simulink model "VCU_Artemiz"  (R2020a)
settings: Solver=FixedStepDiscrete  StartTime=0.0  StopTime=10.0  FixedStep=0.001  RelTol=1e-3  EnableMultiTasking=on
PreLoadFcn:
  | try
  | MDL_setup;
  | catch
  | end
InitFcn:
  | EcoCoder_PreCheckLic();
undefined symbols (not defined in the file): APPS1_max, APPS1_min, APPS2_max, APPS2_min, BRK_TH, DiscIntNeverNeededParam, sigbuilder_block
libraries: CoderSF_BSW_Libs x241, simulink x29
(part 2 of 3)

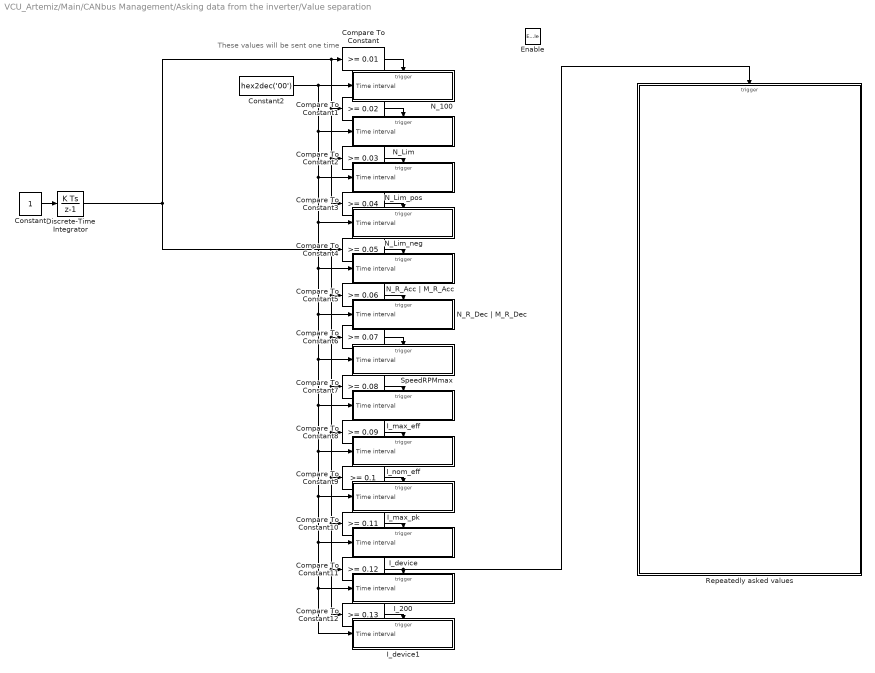
== system VCU_Artemiz/Main/CANbus Management/Asking data from the inverter/Value separation ==
  note: These values will be sent one time
  Enable : EnablePort
  Compare To Constant : simulink/Logic and Bit Operations/Compare To Constant  relop=>=  const=0.01  OutDataTypeStr=boolean
  Compare To Constant1 : simulink/Logic and Bit Operations/Compare To Constant  relop=>=  const=0.02  OutDataTypeStr=boolean
  Compare To Constant10 : simulink/Logic and Bit Operations/Compare To Constant  relop=>=  const=0.11  OutDataTypeStr=boolean
  Compare To Constant11 : simulink/Logic and Bit Operations/Compare To Constant  relop=>=  const=0.12  OutDataTypeStr=boolean
  Compare To Constant12 : simulink/Logic and Bit Operations/Compare To Constant  relop=>=  const=0.13  OutDataTypeStr=boolean
  Compare To Constant2 : simulink/Logic and Bit Operations/Compare To Constant  relop=>=  const=0.03  OutDataTypeStr=boolean
  Compare To Constant3 : simulink/Logic and Bit Operations/Compare To Constant  relop=>=  const=0.04  OutDataTypeStr=boolean
  Compare To Constant4 : simulink/Logic and Bit Operations/Compare To Constant  relop=>=  const=0.05  OutDataTypeStr=boolean
  Compare To Constant5 : simulink/Logic and Bit Operations/Compare To Constant  relop=>=  const=0.06  OutDataTypeStr=boolean
  Compare To Constant6 : simulink/Logic and Bit Operations/Compare To Constant  relop=>=  const=0.07  OutDataTypeStr=boolean
  Compare To Constant7 : simulink/Logic and Bit Operations/Compare To Constant  relop=>=  const=0.08  OutDataTypeStr=boolean
  Compare To Constant8 : simulink/Logic and Bit Operations/Compare To Constant  relop=>=  const=0.09  OutDataTypeStr=boolean
  Compare To Constant9 : simulink/Logic and Bit Operations/Compare To Constant  relop=>=  const=0.1  OutDataTypeStr=boolean
  Constant : Constant  OutDataTypeStr=boolean
  Constant2 : Constant  Value=hex2dec('00')  OutDataTypeStr=uint8
  Discrete-Time Integrator : DiscreteIntegrator  SampleTime=-1  ICPrevOutput=DiscIntNeverNeededParam  ICPrevScaledInput=DiscIntNeverNeededParam
  I_200 : Subsystem
  I_device : Subsystem
  I_device1 : Subsystem
  I_max_eff : Subsystem
  I_max_pk : Subsystem
  I_nom_eff : Subsystem
  N_100 : Subsystem
  N_Lim : Subsystem
  N_Lim_neg : Subsystem
  N_Lim_pos : Subsystem
  N_R_Acc | M_R_Acc : Subsystem
  N_R_Dec | M_R_Dec : Subsystem
  Repeatedly asked values : Subsystem
  SpeedRPMmax : Subsystem
  wires:
  Compare To Constant5/1 -> N_R_Dec | M_R_Dec/Trigger
  Compare To Constant6/1 -> SpeedRPMmax/Trigger
  Compare To Constant4/1 -> N_R_Acc | M_R_Acc/Trigger
  Compare To Constant10/1 -> I_device/Trigger
  Discrete-Time Integrator/1 -> Compare To Constant7/1, Compare To Constant12/1, Compare To Constant11/1, Compare To Constant10/1, Compare To Constant9/1, Compare To Constant8/1, Compare To Constant6/1, Compare To Constant5/1, Compare To Constant4/1, Compare To Constant3/1, Compare To Constant2/1, Compare To Constant1/1, Compare To Constant/1
  Compare To Constant2/1 -> N_Lim_pos/Trigger
  Constant2/1 -> SpeedRPMmax/1(Time interval), I_device1/1(Time interval), I_200/1(Time interval), I_device/1(Time interval), I_max_pk/1(Time interval), I_nom_eff/1(Time interval), I_max_eff/1(Time interval), N_R_Dec | M_R_Dec/1(Time interval), N_R_Acc | M_R_Acc/1(Time interval), N_Lim_neg/1(Time interval), N_Lim_pos/1(Time interval), N_Lim/1(Time interval), N_100/1(Time interval)
  Compare To Constant9/1 -> I_max_pk/Trigger
  Compare To Constant11/1 -> Repeatedly asked values/Trigger, I_200/Trigger
  Compare To Constant/1 -> N_100/Trigger
  Constant/1 -> Discrete-Time Integrator/1
  Compare To Constant7/1 -> I_max_eff/Trigger
  Compare To Constant8/1 -> I_nom_eff/Trigger
  Compare To Constant3/1 -> N_Lim_neg/Trigger
  Compare To Constant1/1 -> N_Lim/Trigger
  Compare To Constant12/1 -> I_device1/Trigger

== system VCU_Artemiz/Main/CANbus Management/Can treatment if len=4 or 5/I_200 ==
  Data : Inport
  Action Port : ActionPort  ActionPortLabel=case [ 217 ]:
  Data Type Conversion : DataTypeConversion
  Write NVM : CoderSF_BSW_Libs/Non-volatile Memory Blocks/Write NVM  variable_name=nvmI_200  flgDef=on  variable_value=0  variable_type=int16  variable_numD=1  unitStr=""  descStr=""  EcoCoderBlockID=N001_NVMVDEF
      settings: AttributesFormatString=value:%<variable_value> type:%<variable_type> D:%<variable_numD>
  Write and Read Measurement : CoderSF_BSW_Libs/Calibration & Measurement/Write and Read Measurement  variable_name=I_200  variable_value=0  variable_type=int16  numD=1  unitStr=""  descStr=""
      settings: AttributesFormatString=type:%<variable_type> Dimensions:%<numD>
  wires:
  Data Type Conversion/1 -> Write and Read Measurement/1
  Write and Read Measurement/1 -> Write NVM/1  "I_200"
  Data/1 -> Data Type Conversion/1

== system VCU_Artemiz/Main/CANbus Management/Can treatment if len=4 or 5/I_act_filt ==
  Data : Inport
  Action Port : ActionPort  ActionPortLabel=case [ 95 ]:
  Data Type Conversion : DataTypeConversion
  Write NVM : CoderSF_BSW_Libs/Non-volatile Memory Blocks/Write NVM  variable_name=nvmI_act_filt  flgDef=on  variable_value=0  variable_type=int16  variable_numD=1  unitStr=""  descStr=""  EcoCoderBlockID=N001_NVMVDEF
      settings: AttributesFormatString=value:%<variable_value> type:%<variable_type> D:%<variable_numD>
  Write and Read Measurement : CoderSF_BSW_Libs/Calibration & Measurement/Write and Read Measurement  variable_name=I_act_filt  variable_value=0  variable_type=int16  numD=1  unitStr=""  descStr=""
      settings: AttributesFormatString=type:%<variable_type> Dimensions:%<numD>
  wires:
  Data Type Conversion/1 -> Write and Read Measurement/1
  Data/1 -> Data Type Conversion/1
  Write and Read Measurement/1 -> Write NVM/1  "I_act_filt"

== system VCU_Artemiz/Main/CANbus Management/Can treatment if len=4 or 5/I_cmd ==
  Data : Inport
  Action Port : ActionPort  ActionPortLabel=case [ 38 ]:
  Data Type Conversion : DataTypeConversion
  Write NVM : CoderSF_BSW_Libs/Non-volatile Memory Blocks/Write NVM  variable_name=nvmI_cmd  flgDef=on  variable_value=0  variable_type=int16  variable_numD=1  unitStr=""  descStr=""  EcoCoderBlockID=N001_NVMVDEF
      settings: AttributesFormatString=value:%<variable_value> type:%<variable_type> D:%<variable_numD>
  Write and Read Measurement : CoderSF_BSW_Libs/Calibration & Measurement/Write and Read Measurement  variable_name=I_cmd  variable_value=0  variable_type=int16  numD=1  unitStr=""  descStr=""
      settings: AttributesFormatString=type:%<variable_type> Dimensions:%<numD>
  wires:
  Data Type Conversion/1 -> Write and Read Measurement/1
  Data/1 -> Data Type Conversion/1
  Write and Read Measurement/1 -> Write NVM/1  "I_cmd"

== system VCU_Artemiz/Main/CANbus Management/Can treatment if len=4 or 5/I_device ==
  Data : Inport
  Action Port : ActionPort  ActionPortLabel=case [ 198 ]:
  Data Type Conversion : DataTypeConversion
  Write NVM : CoderSF_BSW_Libs/Non-volatile Memory Blocks/Write NVM  variable_name=nvmI_device  flgDef=on  variable_value=0  variable_type=int16  variable_numD=1  unitStr=""  descStr=""  EcoCoderBlockID=N001_NVMVDEF
      settings: AttributesFormatString=value:%<variable_value> type:%<variable_type> D:%<variable_numD>
  Write and Read Measurement : CoderSF_BSW_Libs/Calibration & Measurement/Write and Read Measurement  variable_name=I_device  variable_value=0  variable_type=int16  numD=1  unitStr=""  descStr=""
      settings: AttributesFormatString=type:%<variable_type> Dimensions:%<numD>
  wires:
  Data Type Conversion/1 -> Write and Read Measurement/1
  Write and Read Measurement/1 -> Write NVM/1  "I_device"
  Data/1 -> Data Type Conversion/1

== system VCU_Artemiz/Main/CANbus Management/Can treatment if len=4 or 5/I_max_eff ==
  Data : Inport
  Action Port : ActionPort  ActionPortLabel=case [ 77 ]:
  Data Type Conversion : DataTypeConversion
  Write NVM : CoderSF_BSW_Libs/Non-volatile Memory Blocks/Write NVM  variable_name=nvmI_max_eff  flgDef=on  variable_value=0  variable_type=int16  variable_numD=1  unitStr=""  descStr=""  EcoCoderBlockID=N001_NVMVDEF
      settings: AttributesFormatString=value:%<variable_value> type:%<variable_type> D:%<variable_numD>
  Write and Read Measurement : CoderSF_BSW_Libs/Calibration & Measurement/Write and Read Measurement  variable_name=I_max_eff  variable_value=0  variable_type=int16  numD=1  unitStr=""  descStr=""
      settings: AttributesFormatString=type:%<variable_type> Dimensions:%<numD>
  wires:
  Data Type Conversion/1 -> Write and Read Measurement/1
  Data/1 -> Data Type Conversion/1
  Write and Read Measurement/1 -> Write NVM/1  "I_max_eff"

== system VCU_Artemiz/Main/CANbus Management/Can treatment if len=4 or 5/I_max_pk ==
  Data : Inport
  Action Port : ActionPort  ActionPortLabel=case [ 196 ]:
  Data Type Conversion : DataTypeConversion
  Write NVM : CoderSF_BSW_Libs/Non-volatile Memory Blocks/Write NVM  variable_name=nvmI_max_pk  flgDef=on  variable_value=0  variable_type=int16  variable_numD=1  unitStr=""  descStr=""  EcoCoderBlockID=N001_NVMVDEF
      settings: AttributesFormatString=value:%<variable_value> type:%<variable_type> D:%<variable_numD>
  Write and Read Measurement : CoderSF_BSW_Libs/Calibration & Measurement/Write and Read Measurement  variable_name=I_max_pk  variable_value=0  variable_type=int16  numD=1  unitStr=""  descStr=""
      settings: AttributesFormatString=type:%<variable_type> Dimensions:%<numD>
  wires:
  Data Type Conversion/1 -> Write and Read Measurement/1
  Write and Read Measurement/1 -> Write NVM/1  "I_max_pk"
  Data/1 -> Data Type Conversion/1

== system VCU_Artemiz/Main/CANbus Management/Can treatment if len=4 or 5/I_nom_eff ==
  Data : Inport
  Action Port : ActionPort  ActionPortLabel=case [ 78 ]:
  Data Type Conversion : DataTypeConversion
  Write NVM : CoderSF_BSW_Libs/Non-volatile Memory Blocks/Write NVM  variable_name=nvmI_nom_eff  flgDef=on  variable_value=0  variable_type=int16  variable_numD=1  unitStr=""  descStr=""  EcoCoderBlockID=N001_NVMVDEF
      settings: AttributesFormatString=value:%<variable_value> type:%<variable_type> D:%<variable_numD>
  Write and Read Measurement : CoderSF_BSW_Libs/Calibration & Measurement/Write and Read Measurement  variable_name=I_nom_eff  variable_value=0  variable_type=int16  numD=1  unitStr=""  descStr=""
      settings: AttributesFormatString=type:%<variable_type> Dimensions:%<numD>
  wires:
  Data Type Conversion/1 -> Write and Read Measurement/1
  Write and Read Measurement/1 -> Write NVM/1  "I_nom_eff"
  Data/1 -> Data Type Conversion/1

== system VCU_Artemiz/Main/CANbus Management/Can treatment if len=4 or 5/N_100 ==
  Data : Inport
  Action Port : ActionPort  ActionPortLabel=case [ 200 ]:
  Data Type Conversion : DataTypeConversion
  Write NVM : CoderSF_BSW_Libs/Non-volatile Memory Blocks/Write NVM  variable_name=nvmN_100  flgDef=on  variable_value=0  variable_type=uint16  variable_numD=1  unitStr=""  descStr=""  EcoCoderBlockID=N001_NVMVDEF
      settings: AttributesFormatString=value:%<variable_value> type:%<variable_type> D:%<variable_numD>
  Write and Read Measurement : CoderSF_BSW_Libs/Calibration & Measurement/Write and Read Measurement  variable_name=N_100  variable_value=0  variable_type=uint16  numD=1  unitStr=""  descStr=""
      settings: AttributesFormatString=type:%<variable_type> Dimensions:%<numD>
  wires:
  Data Type Conversion/1 -> Write and Read Measurement/1
  Data/1 -> Data Type Conversion/1
  Write and Read Measurement/1 -> Write NVM/1  "N_100"

== system VCU_Artemiz/Main/CANbus Management/Can treatment if len=4 or 5/N_Lim ==
  Data : Inport
  Action Port : ActionPort  ActionPortLabel=case [ 52 ]:
  Data Type Conversion : DataTypeConversion
  Write NVM : CoderSF_BSW_Libs/Non-volatile Memory Blocks/Write NVM  variable_name=nvmN_lim  flgDef=on  variable_value=0  variable_type=uint16  variable_numD=1  unitStr=""  descStr=""  EcoCoderBlockID=N001_NVMVDEF
      settings: AttributesFormatString=value:%<variable_value> type:%<variable_type> D:%<variable_numD>
  Write and Read Measurement : CoderSF_BSW_Libs/Calibration & Measurement/Write and Read Measurement  variable_name=N_lim  variable_value=0  variable_type=uint16  numD=1  unitStr=""  descStr=""
      settings: AttributesFormatString=type:%<variable_type> Dimensions:%<numD>
  wires:
  Data Type Conversion/1 -> Write and Read Measurement/1
  Data/1 -> Data Type Conversion/1
  Write and Read Measurement/1 -> Write NVM/1  "N_lim"

== system VCU_Artemiz/Main/CANbus Management/Can treatment if len=4 or 5/N_Lim_neg ==
  Data : Inport
  Action Port : ActionPort  ActionPortLabel=case [ 62 ]:
  Data Type Conversion : DataTypeConversion
  Write NVM : CoderSF_BSW_Libs/Non-volatile Memory Blocks/Write NVM  variable_name=nvmN_lim_neg  flgDef=on  variable_value=0  variable_type=int16  variable_numD=1  unitStr=""  descStr=""  EcoCoderBlockID=N001_NVMVDEF
      settings: AttributesFormatString=value:%<variable_value> type:%<variable_type> D:%<variable_numD>
  Write and Read Measurement : CoderSF_BSW_Libs/Calibration & Measurement/Write and Read Measurement  variable_name=N_lim_neg  variable_value=0  variable_type=int16  numD=1  unitStr=""  descStr=""
      settings: AttributesFormatString=type:%<variable_type> Dimensions:%<numD>
  wires:
  Data Type Conversion/1 -> Write and Read Measurement/1
  Data/1 -> Data Type Conversion/1
  Write and Read Measurement/1 -> Write NVM/1  "N_lim_neg"

== system VCU_Artemiz/Main/CANbus Management/Can treatment if len=4 or 5/N_Lim_pos ==
  Data : Inport
  Action Port : ActionPort  ActionPortLabel=case [ 63 ]:
  Data Type Conversion : DataTypeConversion
  Write NVM : CoderSF_BSW_Libs/Non-volatile Memory Blocks/Write NVM  variable_name=nvmN_lim_pos  flgDef=on  variable_value=0  variable_type=int16  variable_numD=1  unitStr=""  descStr=""  EcoCoderBlockID=N001_NVMVDEF
      settings: AttributesFormatString=value:%<variable_value> type:%<variable_type> D:%<variable_numD>
  Write and Read Measurement : CoderSF_BSW_Libs/Calibration & Measurement/Write and Read Measurement  variable_name=N_lim_pos  variable_value=0  variable_type=int16  numD=1  unitStr=""  descStr=""
      settings: AttributesFormatString=type:%<variable_type> Dimensions:%<numD>
  wires:
  Data Type Conversion/1 -> Write and Read Measurement/1
  Data/1 -> Data Type Conversion/1
  Write and Read Measurement/1 -> Write NVM/1  "N_lim_pos"

== system VCU_Artemiz/Main/CANbus Management/Can treatment if len=4 or 5/N_act_filt ==
  Data : Inport
  Action Port : ActionPort  ActionPortLabel=case [ 168 ]:
  Data Type Conversion : DataTypeConversion
  Write NVM : CoderSF_BSW_Libs/Non-volatile Memory Blocks/Write NVM  variable_name=nvmN_act_filt  flgDef=on  variable_value=0  variable_type=int16  variable_numD=1  unitStr=""  descStr=""  EcoCoderBlockID=N001_NVMVDEF
      settings: AttributesFormatString=value:%<variable_value> type:%<variable_type> D:%<variable_numD>
  Write and Read Measurement : CoderSF_BSW_Libs/Calibration & Measurement/Write and Read Measurement  variable_name=N_act_filt  variable_value=0  variable_type=int16  numD=1  unitStr=""  descStr=""
      settings: AttributesFormatString=type:%<variable_type> Dimensions:%<numD>
  wires:
  Data Type Conversion/1 -> Write and Read Measurement/1
  Write and Read Measurement/1 -> Write NVM/1  "N_act_filt"
  Data/1 -> Data Type Conversion/1

== system VCU_Artemiz/Main/CANbus Management/Can treatment if len=4 or 5/SpeedRPMmax ==
  Data : Inport
  Action Port : ActionPort  ActionPortLabel=case [ 206 ]:
  Data Type Conversion : DataTypeConversion
  Write NVM : CoderSF_BSW_Libs/Non-volatile Memory Blocks/Write NVM  variable_name=nvmSpeedRPMmax  flgDef=on  variable_value=0  variable_type=int16  variable_numD=1  unitStr=""  descStr=""  EcoCoderBlockID=N001_NVMVDEF
      settings: AttributesFormatString=value:%<variable_value> type:%<variable_type> D:%<variable_numD>
  Write and Read Measurement : CoderSF_BSW_Libs/Calibration & Measurement/Write and Read Measurement  variable_name=SpeedRPMmax  variable_value=0  variable_type=int16  numD=1  unitStr=""  descStr=""
      settings: AttributesFormatString=type:%<variable_type> Dimensions:%<numD>
  wires:
  Data Type Conversion/1 -> Write and Read Measurement/1
  Write and Read Measurement/1 -> Write NVM/1  "SpeedRPMmax"
  Data/1 -> Data Type Conversion/1

== system VCU_Artemiz/Main/CANbus Management/Can treatment if len=4 or 5/T_IGBT ==
  Data : Inport
  Action Port : ActionPort  ActionPortLabel=case [ 74 ]:
  Data Type Conversion : DataTypeConversion
  Write NVM : CoderSF_BSW_Libs/Non-volatile Memory Blocks/Write NVM  variable_name=nvmT_IGBT  flgDef=on  variable_value=0  variable_type=int16  variable_numD=1  unitStr=""  descStr=""  EcoCoderBlockID=N001_NVMVDEF
      settings: AttributesFormatString=value:%<variable_value> type:%<variable_type> D:%<variable_numD>
  Write and Read Measurement : CoderSF_BSW_Libs/Calibration & Measurement/Write and Read Measurement  variable_name=T_IGBT  variable_value=0  variable_type=int16  numD=1  unitStr=""  descStr=""
      settings: AttributesFormatString=type:%<variable_type> Dimensions:%<numD>
  wires:
  Data Type Conversion/1 -> Write and Read Measurement/1
  Data/1 -> Data Type Conversion/1
  Write and Read Measurement/1 -> Write NVM/1  "T_IGBT"

== system VCU_Artemiz/Main/CANbus Management/Can treatment if len=4 or 5/T_air ==
  Data : Inport
  Action Port : ActionPort  ActionPortLabel=case [ 75 ]:
  Data Type Conversion : DataTypeConversion
  Write NVM : CoderSF_BSW_Libs/Non-volatile Memory Blocks/Write NVM  variable_name=nvmT_air  flgDef=on  variable_value=0  variable_type=int16  variable_numD=1  unitStr=""  descStr=""  EcoCoderBlockID=N001_NVMVDEF
      settings: AttributesFormatString=value:%<variable_value> type:%<variable_type> D:%<variable_numD>
  Write and Read Measurement : CoderSF_BSW_Libs/Calibration & Measurement/Write and Read Measurement  variable_name=T_air  variable_value=0  variable_type=int16  numD=1  unitStr=""  descStr=""
      settings: AttributesFormatString=type:%<variable_type> Dimensions:%<numD>
  wires:
  Data Type Conversion/1 -> Write and Read Measurement/1
  Data/1 -> Data Type Conversion/1
  Write and Read Measurement/1 -> Write NVM/1  "T_air"

== system VCU_Artemiz/Main/CANbus Management/Can treatment if len=4 or 5/T_motor ==
  Data : Inport
  Action Port : ActionPort  ActionPortLabel=case [ 73 ]:
  Data Type Conversion : DataTypeConversion
  Write NVM : CoderSF_BSW_Libs/Non-volatile Memory Blocks/Write NVM  variable_name=nvmT_motor  flgDef=on  variable_value=0  variable_type=int16  variable_numD=1  unitStr=""  descStr=""  EcoCoderBlockID=N001_NVMVDEF
      settings: AttributesFormatString=value:%<variable_value> type:%<variable_type> D:%<variable_numD>
  Write and Read Measurement : CoderSF_BSW_Libs/Calibration & Measurement/Write and Read Measurement  variable_name=T_motor  variable_value=0  variable_type=int16  numD=1  unitStr=""  descStr=""
      settings: AttributesFormatString=type:%<variable_type> Dimensions:%<numD>
  wires:
  Data Type Conversion/1 -> Write and Read Measurement/1
  Data/1 -> Data Type Conversion/1
  Write and Read Measurement/1 -> Write NVM/1  "T_motor"

== system VCU_Artemiz/Main/CANbus Management/Can treatment if len=4 or 5/Vdc_bus ==
  Data : Inport
  Action Port : ActionPort  ActionPortLabel=case [ 235 ]:
  Data Type Conversion : DataTypeConversion
  Write NVM : CoderSF_BSW_Libs/Non-volatile Memory Blocks/Write NVM  variable_name=nvmVdc_bus  flgDef=on  variable_value=0  variable_type=int16  variable_numD=1  unitStr=""  descStr=""  EcoCoderBlockID=N001_NVMVDEF
      settings: AttributesFormatString=value:%<variable_value> type:%<variable_type> D:%<variable_numD>
  Write and Read Measurement : CoderSF_BSW_Libs/Calibration & Measurement/Write and Read Measurement  variable_name=Vdc_bus  variable_value=0  variable_type=int16  numD=1  unitStr=""  descStr=""
      settings: AttributesFormatString=type:%<variable_type> Dimensions:%<numD>
  wires:
  Data Type Conversion/1 -> Write and Read Measurement/1
  Data/1 -> Data Type Conversion/1
  Write and Read Measurement/1 -> Write NVM/1  "Vdc_bus"

== system VCU_Artemiz/Main/CANbus Management/Can treatment if len=6/N_R_Acc | M R_Acc ==
  Data : Inport
  Action Port : ActionPort  ActionPortLabel=case [ 53 ]:
  Data Type Conversion1 : DataTypeConversion  OutDataTypeStr=int16
  Data Type Conversion2 : DataTypeConversion  OutDataTypeStr=int16
  Extract Bits : simulink/Logic and Bit Operations/Extract Bits  bitsToExtract=Lower half  numBits=8  bitIdxRange=[0 7]  outScalingMode=Treat bit field as an integer
  Extract Bits1 : simulink/Logic and Bit Operations/Extract Bits  bitsToExtract=Upper half  numBits=8  bitIdxRange=[0 7]  outScalingMode=Treat bit field as an integer
  Write NVM : CoderSF_BSW_Libs/Non-volatile Memory Blocks/Write NVM  variable_name=nvmN_R_Acc  flgDef=on  variable_value=0  variable_type=int16  variable_numD=1  unitStr=""  descStr=""  EcoCoderBlockID=N001_NVMVDEF
      settings: AttributesFormatString=value:%<variable_value> type:%<variable_type> D:%<variable_numD>
  Write NVM1 : CoderSF_BSW_Libs/Non-volatile Memory Blocks/Write NVM  variable_name=nvmM_R_Acc  flgDef=on  variable_value=0  variable_type=int16  variable_numD=1  unitStr=""  descStr=""  EcoCoderBlockID=N001_NVMVDEF
      settings: AttributesFormatString=value:%<variable_value> type:%<variable_type> D:%<variable_numD>
  Write and Read Measurement : CoderSF_BSW_Libs/Calibration & Measurement/Write and Read Measurement  variable_name=N_R_Acc  variable_value=0  variable_type=int16  numD=1  unitStr=""  descStr=""
      settings: AttributesFormatString=type:%<variable_type> Dimensions:%<numD>
  Write and Read Measurement1 : CoderSF_BSW_Libs/Calibration & Measurement/Write and Read Measurement  variable_name=M_R_Acc  variable_value=0  variable_type=int16  numD=1  unitStr=""  descStr=""
      settings: AttributesFormatString=type:%<variable_type> Dimensions:%<numD>
  wires:
  Data/1 -> Extract Bits1/1, Extract Bits/1
  Extract Bits/1 -> Data Type Conversion2/1
  Data Type Conversion2/1 -> Write and Read Measurement/1
  Extract Bits1/1 -> Data Type Conversion1/1
  Data Type Conversion1/1 -> Write and Read Measurement1/1
  Write and Read Measurement/1 -> Write NVM/1  "N_R_Acc"
  Write and Read Measurement1/1 -> Write NVM1/1  "M_R_Acc"

== system VCU_Artemiz/Main/CANbus Management/Can treatment if len=6/N_R_Dec | M_R_Dec ==
  Data : Inport
  Action Port : ActionPort  ActionPortLabel=case [ 237 ]:
  Data Type Conversion1 : DataTypeConversion  OutDataTypeStr=int16
  Data Type Conversion2 : DataTypeConversion  OutDataTypeStr=int16
  Extract Bits : simulink/Logic and Bit Operations/Extract Bits  bitsToExtract=Lower half  numBits=8  bitIdxRange=[0 7]  outScalingMode=Treat bit field as an integer
  Extract Bits1 : simulink/Logic and Bit Operations/Extract Bits  bitsToExtract=Upper half  numBits=8  bitIdxRange=[0 7]  outScalingMode=Treat bit field as an integer
  Write NVM : CoderSF_BSW_Libs/Non-volatile Memory Blocks/Write NVM  variable_name=nvmN_R_Dec  flgDef=on  variable_value=0  variable_type=int16  variable_numD=1  unitStr=""  descStr=""  EcoCoderBlockID=N001_NVMVDEF
      settings: AttributesFormatString=value:%<variable_value> type:%<variable_type> D:%<variable_numD>
  Write NVM1 : CoderSF_BSW_Libs/Non-volatile Memory Blocks/Write NVM  variable_name=nvmM_R_Dec  flgDef=on  variable_value=0  variable_type=int16  variable_numD=1  unitStr=""  descStr=""  EcoCoderBlockID=N001_NVMVDEF
      settings: AttributesFormatString=value:%<variable_value> type:%<variable_type> D:%<variable_numD>
  Write and Read Measurement : CoderSF_BSW_Libs/Calibration & Measurement/Write and Read Measurement  variable_name=N_R_Dec  variable_value=0  variable_type=int16  numD=1  unitStr=""  descStr=""
      settings: AttributesFormatString=type:%<variable_type> Dimensions:%<numD>
  Write and Read Measurement1 : CoderSF_BSW_Libs/Calibration & Measurement/Write and Read Measurement  variable_name=M_R_Dec  variable_value=0  variable_type=int16  numD=1  unitStr=""  descStr=""
      settings: AttributesFormatString=type:%<variable_type> Dimensions:%<numD>
  wires:
  Data Type Conversion2/1 -> Write and Read Measurement/1
  Data Type Conversion1/1 -> Write and Read Measurement1/1
  Data/1 -> Extract Bits1/1, Extract Bits/1
  Extract Bits1/1 -> Data Type Conversion1/1
  Extract Bits/1 -> Data Type Conversion2/1
  Write and Read Measurement/1 -> Write NVM/1  "N_R_Dec"
  Write and Read Measurement1/1 -> Write NVM1/1  "M_R_Dec"

== system VCU_Artemiz/Main/CANbus Management/Initialization/Disabling the inverter ==
  Constant : Constant  Value=hex2dec('51')  OutDataTypeStr=uint8
  Constant1 : Constant  Value=hex2dec('0004')  OutDataTypeStr=uint16
  Pack Signals To CAN Data : CoderSF_BSW_Libs/CAN/Pack Signals To CAN Data  Signal="{{'REG_ID'  'Data1'},[0 8],[8 16],{'uint8'  'uint16'},{'Intel' 'Intel'}}"
  Send CAN Data : CoderSF_BSW_Libs/CAN/Send CAN Data  channel=CAN_A  txlen=3  txid=hex2dec('201')  frametype=Standard(11-bit ID)  showerror=off
  wires:
  Constant/1 -> Pack Signals To CAN Data/1
  Pack Signals To CAN Data/1 -> Send CAN Data/1
  Constant1/1 -> Pack Signals To CAN Data/2

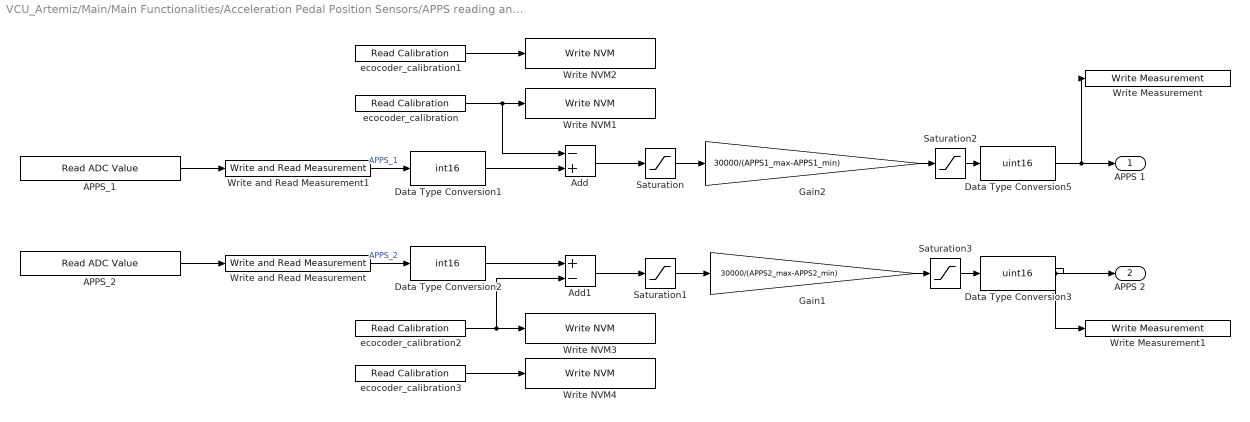
== system VCU_Artemiz/Main/Main Functionalities/Acceleration Pedal Position Sensors/APPS reading and calibration ==
  APPS_1 : CoderSF_BSW_Libs/ADC/Read ADC Value  channel=3
  APPS_2 : CoderSF_BSW_Libs/ADC/Read ADC Value  channel=4
  Add : Sum  Inputs=-+
  Add1 : Sum  Inputs=+-
  Data Type Conversion1 : DataTypeConversion  OutDataTypeStr=int16
  Data Type Conversion2 : DataTypeConversion  OutDataTypeStr=int16
  Data Type Conversion3 : DataTypeConversion  OutDataTypeStr=uint16
  Data Type Conversion5 : DataTypeConversion  OutDataTypeStr=uint16
  Gain1 : Gain  Gain=30000/(APPS2_max-APPS2_min)  OutDataTypeStr=int32
  Gain2 : Gain  Gain=30000/(APPS1_max-APPS1_min)  OutDataTypeStr=int32
  Saturation : Saturate  UpperLimit=4095  LowerLimit=0  OutDataTypeStr=int16
  Saturation1 : Saturate  UpperLimit=4095  LowerLimit=0  OutDataTypeStr=int16
  Saturation2 : Saturate  UpperLimit=30000  LowerLimit=0  OutDataTypeStr=int32
  Saturation3 : Saturate  UpperLimit=30000  LowerLimit=0  OutDataTypeStr=int32
  Write Measurement : CoderSF_BSW_Libs/Calibration & Measurement/Write Measurement  variable_name=APPS1_calib  variable_value=0  variable_type=uint16  numD=1  unitStr=""  descStr=""
      settings: AttributesFormatString=type:%<variable_type> Dimensions:%<numD>
  Write Measurement1 : CoderSF_BSW_Libs/Calibration & Measurement/Write Measurement  variable_name=APPS2_calib  variable_value=0  variable_type=uint16  numD=1  unitStr=""  descStr=""
      settings: AttributesFormatString=type:%<variable_type> Dimensions:%<numD>
  Write NVM1 : CoderSF_BSW_Libs/Non-volatile Memory Blocks/Write NVM  variable_name=nvmAPPS1_min  flgDef=on  variable_value=0  variable_type=int16  variable_numD=1  unitStr=""  descStr=""  EcoCoderBlockID=N001_NVMVDEF
      settings: AttributesFormatString=value:%<variable_value> type:%<variable_type> D:%<variable_numD>
  Write NVM2 : CoderSF_BSW_Libs/Non-volatile Memory Blocks/Write NVM  variable_name=nvmAPPS1_max  flgDef=on  variable_value=0  variable_type=int16  variable_numD=1  unitStr=""  descStr=""  EcoCoderBlockID=N001_NVMVDEF
      settings: AttributesFormatString=value:%<variable_value> type:%<variable_type> D:%<variable_numD>
  Write NVM3 : CoderSF_BSW_Libs/Non-volatile Memory Blocks/Write NVM  variable_name=nvmAPPS2_min  flgDef=on  variable_value=0  variable_type=int16  variable_numD=1  unitStr=""  descStr=""  EcoCoderBlockID=N001_NVMVDEF
      settings: AttributesFormatString=value:%<variable_value> type:%<variable_type> D:%<variable_numD>
  Write NVM4 : CoderSF_BSW_Libs/Non-volatile Memory Blocks/Write NVM  variable_name=nvmAPPS2_max  flgDef=on  variable_value=0  variable_type=int16  variable_numD=1  unitStr=""  descStr=""  EcoCoderBlockID=N001_NVMVDEF
      settings: AttributesFormatString=value:%<variable_value> type:%<variable_type> D:%<variable_numD>
  Write and Read Measurement : CoderSF_BSW_Libs/Calibration & Measurement/Write and Read Measurement  variable_name=APPS_2  variable_value=0  variable_type=uint16  numD=1  unitStr=""  descStr=""
      settings: AttributesFormatString=type:%<variable_type> Dimensions:%<numD>
  Write and Read Measurement1 : CoderSF_BSW_Libs/Calibration & Measurement/Write and Read Measurement  variable_name=APPS_1  variable_value=0  variable_type=uint16  numD=1  unitStr=""  descStr=""
      settings: AttributesFormatString=type:%<variable_type> Dimensions:%<numD>
  ecocoder_calibration : CoderSF_BSW_Libs/Calibration & Measurement/Read Calibration  variable_name=APPS1_min  variable_value=750  variable_type=int16  variable_min=[]  variable_max=[]  unitStr=""  descStr=""
      settings: AttributesFormatString=value:%<variable_value> type:%<variable_type> max:%<variable_max> Min:%<variable_min>
  ecocoder_calibration1 : CoderSF_BSW_Libs/Calibration & Measurement/Read Calibration  variable_name=APPS1_max  variable_value=1293  variable_type=int16  variable_min=[]  variable_max=[]  unitStr=""  descStr=""
      settings: AttributesFormatString=value:%<variable_value> type:%<variable_type> max:%<variable_max> Min:%<variable_min>
  ecocoder_calibration2 : CoderSF_BSW_Libs/Calibration & Measurement/Read Calibration  variable_name=APPS2_min  variable_value=366  variable_type=int16  variable_min=[]  variable_max=[]  unitStr=""  descStr=""
      settings: AttributesFormatString=value:%<variable_value> type:%<variable_type> max:%<variable_max> Min:%<variable_min>
  ecocoder_calibration3 : CoderSF_BSW_Libs/Calibration & Measurement/Read Calibration  variable_name=APPS2_max  variable_value=912  variable_type=int16  variable_min=[]  variable_max=[]  unitStr=""  descStr=""
      settings: AttributesFormatString=value:%<variable_value> type:%<variable_type> max:%<variable_max> Min:%<variable_min>
  APPS 1 : Outport
  APPS 2 : Outport  Port=2
  wires:
  APPS_2/1 -> Write and Read Measurement/1
  Write and Read Measurement1/1 -> Data Type Conversion1/1  "APPS_1"
  Write and Read Measurement/1 -> Data Type Conversion2/1  "APPS_2"
  APPS_1/1 -> Write and Read Measurement1/1
  Saturation/1 -> Gain2/1
  Data Type Conversion5/1 -> Write Measurement/1, APPS 1/1
  ecocoder_calibration/1 -> Add/1, Write NVM1/1
  ecocoder_calibration1/1 -> Write NVM2/1
  ecocoder_calibration2/1 -> Add1/2, Write NVM3/1
  ecocoder_calibration3/1 -> Write NVM4/1
  Data Type Conversion1/1 -> Add/2
  Add/1 -> Saturation/1
  Add1/1 -> Saturation1/1
  Saturation1/1 -> Gain1/1
  Data Type Conversion3/1 -> Write Measurement1/1, APPS 2/1
  Data Type Conversion2/1 -> Add1/1
  Gain2/1 -> Saturation2/1
  Saturation2/1 -> Data Type Conversion5/1
  Gain1/1 -> Saturation3/1
  Saturation3/1 -> Data Type Conversion3/1

== system VCU_Artemiz/Main/Main Functionalities/Acceleration Pedal Position Sensors/Check APPS Implausibility ==
  note: Check if the implausibility persists for more than 100ms
  note: Check if there is an APPS implausibility (T 11.8.9)
  APPS 1 : Inport
  APPS 2 : Inport  Port=2
  Abs : Abs  OutDataTypeStr=uint16
  Compare To Constant : simulink/Logic and Bit Operations/Compare To Constant  relop=>=  const=30000  OutDataTypeStr=boolean
  Compare To Constant1 : simulink/Logic and Bit Operations/Compare To Constant  relop=>=  const=0.1  OutDataTypeStr=boolean
  Discrete-Time Integrator : DiscreteIntegrator  ExternalReset=falling  SampleTime=-1  OutDataTypeStr=Inherit: Inherit via back propagation  UpperSaturationLimit=12  ICPrevOutput=DiscIntNeverNeededParam  ICPrevScaledInput=DiscIntNeverNeededParam
  Gain1 : Gain  Gain=10  OutDataTypeStr=uint32
  Subtract : Sum  Inputs=+-  OutDataTypeStr=int16
  Write Measurement : CoderSF_BSW_Libs/Calibration & Measurement/Write Measurement  variable_name=APPS_PBM  variable_value=0  variable_type=boolean  numD=1  unitStr=""  descStr=""
      settings: AttributesFormatString=type:%<variable_type> Dimensions:%<numD>
  Write Measurement2 : CoderSF_BSW_Libs/Calibration & Measurement/Write Measurement  variable_name=APPS_implausibility  variable_value=0  variable_type=boolean  numD=1  unitStr=""  descStr=""
      settings: AttributesFormatString=type:%<variable_type> Dimensions:%<numD>
  Write NVM4 : CoderSF_BSW_Libs/Non-volatile Memory Blocks/Write NVM  variable_name=nvmAPPS_PBM  flgDef=on  variable_value=0  variable_type=boolean  variable_numD=1  unitStr=""  descStr=""  EcoCoderBlockID=N001_NVMVDEF
      settings: AttributesFormatString=value:%<variable_value> type:%<variable_type> D:%<variable_numD>
  tag scope: APPS_PBM=global
  wires:
  Discrete-Time Integrator/1 -> Compare To Constant1/1
  Subtract/1 -> Abs/1
  Compare To Constant/1 -> Write Measurement2/1, Discrete-Time Integrator/2, Discrete-Time Integrator/1
  APPS 2/1 -> Subtract/2
  Abs/1 -> Gain1/1
  Compare To Constant1/1 -> [APPS_PBM], Write Measurement/1, Write NVM4/1  "APPS_PBM"
  Gain1/1 -> Compare To Constant/1
  APPS 1/1 -> Subtract/1

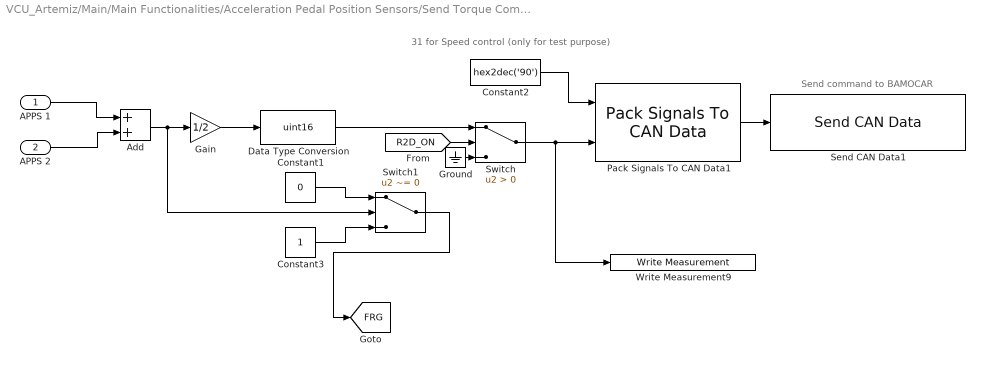
== system VCU_Artemiz/Main/Main Functionalities/Acceleration Pedal Position Sensors/Send Torque Command ==
  note: 31 for Speed control (only for test purpose)
  note: Send command to BAMOCAR
  APPS 1 : Inport
  APPS 2 : Inport  Port=2
  Add : Sum  OutDataTypeStr=uint32
  Constant1 : Constant  Value=0  OutDataTypeStr=boolean
  Constant2 : Constant  Value=hex2dec('90')  OutDataTypeStr=uint8
  Constant3 : Constant  OutDataTypeStr=boolean
  Data Type Conversion : DataTypeConversion  OutDataTypeStr=uint16
  Gain : Gain  Gain=1/2
  Ground : Ground
  Pack Signals To CAN Data1 : CoderSF_BSW_Libs/CAN/Pack Signals To CAN Data  Signal="{{'REG_90'  'Data1'},[0 8],[8 24],{'uint8'  'uint16'},{'Intel' 'Intel'}}"
  Send CAN Data1 : CoderSF_BSW_Libs/CAN/Send CAN Data  channel=CAN_A  txlen=3  txid="hex2dec(\"201\")"  frametype=Standard(11-bit ID)  showerror=off
  Switch : Switch  Criteria=u2 > Threshold
  Switch1 : Switch  Criteria=u2 ~= 0  Threshold=1
  Write Measurement9 : CoderSF_BSW_Libs/Calibration & Measurement/Write Measurement  variable_name=TRQ_CMD_BAMOCAR  variable_value=0  variable_type=uint16  numD=1  unitStr=""  descStr=""
      settings: AttributesFormatString=type:%<variable_type> Dimensions:%<numD>
  tag scope: FRG=global
  wires:
  Pack Signals To CAN Data1/1 -> Send CAN Data1/1
  Gain/1 -> Data Type Conversion/1
  APPS 2/1 -> Add/2
  APPS 1/1 -> Add/1
  Constant2/1 -> Pack Signals To CAN Data1/1
  [R2D_ON] -> Switch/2
  Switch/1 -> Write Measurement9/1, Pack Signals To CAN Data1/2
  Ground/1 -> Switch/3
  Data Type Conversion/1 -> Switch/1
  Add/1 -> Switch1/2, Gain/1
  Constant1/1 -> Switch1/1
  Constant3/1 -> Switch1/3
  Switch1/1 -> [FRG]

== system VCU_Artemiz/Main/Main Functionalities/Ready to drive/Enable Inverter ==
  Trigger : TriggerPort  TriggerType=either  VariantControl=Variant  PortDimensions=1
  Constant : Constant  Value=hex2dec('51')  OutDataTypeStr=uint8
  Constant1 : Constant  Value=hex2dec('0000')  OutDataTypeStr=uint16
  Pack Signals To CAN Data : CoderSF_BSW_Libs/CAN/Pack Signals To CAN Data  Signal="{{'REG_ID'  'Data1'},[0 8],[8 16],{'uint8'  'uint16'},{'Intel' 'Intel'}}"
  Send CAN Data : CoderSF_BSW_Libs/CAN/Send CAN Data  channel=CAN_A  txlen=3  txid=hex2dec('201')  frametype=Standard(11-bit ID)  showerror=off
  wires:
  Constant/1 -> Pack Signals To CAN Data/1
  Pack Signals To CAN Data/1 -> Send CAN Data/1
  Constant1/1 -> Pack Signals To CAN Data/2

== system VCU_Artemiz/Main/Main Functionalities/Ready to drive/Subsystem ==
  note: Must press during 1s
  Compare To Constant3 : simulink/Logic and Bit Operations/Compare To Constant  relop=>=  const=1  OutDataTypeStr=boolean
  Discrete-Time Integrator1 : DiscreteIntegrator  ExternalReset=falling  SampleTime=-1  OutDataTypeStr=Inherit: Inherit via back propagation  UpperSaturationLimit=12  ICPrevOutput=DiscIntNeverNeededParam  ICPrevScaledInput=DiscIntNeverNeededParam
  FLWS : CoderSF_BSW_Libs/Digital I//O/Switch Input  portNum=DI32
  Logical Operator : Logic  AllPortsSameDT=off  OutDataTypeStr=boolean
  R2D Button : CoderSF_BSW_Libs/Digital I//O/Switch Input  portNum=DI13
  Write Measurement1 : CoderSF_BSW_Libs/Calibration & Measurement/Write Measurement  variable_name=FLWS  variable_value=0  variable_type=boolean  numD=1  unitStr=""  descStr=""
      settings: AttributesFormatString=type:%<variable_type> Dimensions:%<numD>
  Write Measurement6 : CoderSF_BSW_Libs/Calibration & Measurement/Write Measurement  variable_name=R2D_btn  variable_value=0  variable_type=boolean  numD=1  unitStr=""  descStr=""
      settings: AttributesFormatString=type:%<variable_type> Dimensions:%<numD>
  R2D_ASKED : Outport
  wires:
  Logical Operator/1 -> Discrete-Time Integrator1/1, Discrete-Time Integrator1/2
  Discrete-Time Integrator1/1 -> Compare To Constant3/1
  [BRAKE_ON] -> Logical Operator/1
  Compare To Constant3/1 -> R2D_ASKED/1
  R2D Button/1 -> Logical Operator/2, Write Measurement6/1
  FLWS/1 -> Write Measurement1/1

== system VCU_Artemiz/Main/Main Functionalities/Ready to drive/Subsystem1 ==
  Trigger : Inport
  Exit : Inport  Port=2
  Compare To Constant5 : simulink/Logic and Bit Operations/Compare To Constant  relop=<=  const=2  OutDataTypeStr=boolean
  Compare To Constant7 : simulink/Logic and Bit Operations/Compare To Constant  relop=>  const=0.1  OutDataTypeStr=boolean
  Discrete-Time Integrator2 : DiscreteIntegrator  ExternalReset=falling  SampleTime=-1  OutDataTypeStr=Inherit: Inherit via back propagation  UpperSaturationLimit=12  ICPrevOutput=DiscIntNeverNeededParam  ICPrevScaledInput=DiscIntNeverNeededParam
  Enter R2D Mode : Subsystem  TreatAsAtomicUnit=on
  Logical Operator5 : Logic  IconShape=distinctive  AllPortsSameDT=off  OutDataTypeStr=boolean
  R2D LED : CoderSF_BSW_Libs/Digital I//O/Switch Output  channel=LSO03
  R2D Sound : CoderSF_BSW_Libs/Digital I//O/Switch Output  channel=LSO01
  Write Measurement : CoderSF_BSW_Libs/Calibration & Measurement/Write Measurement  variable_name=R2D  variable_value=0  variable_type=boolean  numD=1  unitStr=""  descStr=""
      settings: AttributesFormatString=type:%<variable_type> Dimensions:%<numD>
  Write Measurement3 : CoderSF_BSW_Libs/Calibration & Measurement/Write Measurement  variable_name=BUZZ  variable_value=0  variable_type=boolean  numD=1  unitStr=""  descStr=""
      settings: AttributesFormatString=type:%<variable_type> Dimensions:%<numD>
  Write NVM : CoderSF_BSW_Libs/Non-volatile Memory Blocks/Write NVM  variable_name=nvm_R2D  flgDef=on  variable_value=0  variable_type=boolean  variable_numD=1  unitStr=""  descStr=""  EcoCoderBlockID=N001_NVMVDEF
      settings: AttributesFormatString=value:%<variable_value> type:%<variable_type> D:%<variable_numD>
  tag scope: R2D_ON=global
  wires:
  Trigger/1 -> Enter R2D Mode/Trigger
  Exit/1 -> Enter R2D Mode/1(Exit)
  Compare To Constant5/1 -> Logical Operator5/2
  Compare To Constant7/1 -> Logical Operator5/1
  Enter R2D Mode/1(R2D Sound) -> Discrete-Time Integrator2/1, Discrete-Time Integrator2/2
  Discrete-Time Integrator2/1 -> Compare To Constant7/1, Compare To Constant5/1
  Logical Operator5/1 -> R2D Sound/1, Write Measurement3/1
  Enter R2D Mode/2(R2D Led) -> R2D LED/1, Write NVM/1, Write Measurement/1, [R2D_ON]

== system VCU_Artemiz/Main/Main Functionalities/Tractive System/Subsystem ==
  note: Must press during 1s
  Compare To Constant3 : simulink/Logic and Bit Operations/Compare To Constant  relop=>=  const=1  OutDataTypeStr=boolean
  Discrete-Time Integrator1 : DiscreteIntegrator  ExternalReset=falling  SampleTime=-1  OutDataTypeStr=Inherit: Inherit via back propagation  UpperSaturationLimit=12  ICPrevOutput=DiscIntNeverNeededParam  ICPrevScaledInput=DiscIntNeverNeededParam
  Pump2 : CoderSF_BSW_Libs/Digital I//O/Switch Output  channel=LSO06
  Subsystem : Subsystem
  TS Button : CoderSF_BSW_Libs/Digital I//O/Switch Input  portNum=DI09
  Write Measurement : CoderSF_BSW_Libs/Calibration & Measurement/Write Measurement  variable_name=TS  variable_value=0  variable_type=boolean  numD=1  unitStr=""  descStr=""
      settings: AttributesFormatString=type:%<variable_type> Dimensions:%<numD>
  Write Measurement1 : CoderSF_BSW_Libs/Calibration & Measurement/Write Measurement  variable_name=TSBTN  variable_value=0  variable_type=boolean  numD=1  unitStr=""  descStr=""
      settings: AttributesFormatString=type:%<variable_type> Dimensions:%<numD>
  Write NVM : CoderSF_BSW_Libs/Non-volatile Memory Blocks/Write NVM  variable_name=nvm_TS_ON  flgDef=on  variable_value=false  variable_type=boolean  variable_numD=1  unitStr=""  descStr=""  EcoCoderBlockID=N001_NVMVDEF
      settings: AttributesFormatString=value:%<variable_value> type:%<variable_type> D:%<variable_numD>
  TS ON : Outport
  tag scope: TS_ON=global
  wires:
  Discrete-Time Integrator1/1 -> Compare To Constant3/1
  Compare To Constant3/1 -> Subsystem/Trigger, Subsystem/1(In1)
  Subsystem/1(TS ON) -> Write Measurement/1, Write NVM/1, Pump2/1, TS ON/1, [TS_ON]
  TS Button/1 -> Discrete-Time Integrator1/1, Discrete-Time Integrator1/2, Write Measurement1/1

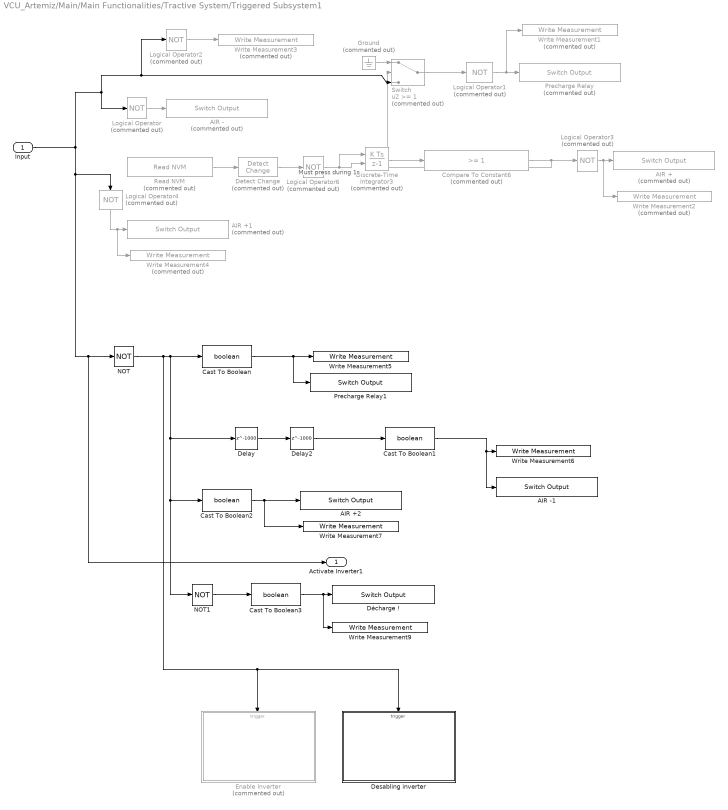
== system VCU_Artemiz/Main/Main Functionalities/Tractive System/Triggered Subsystem1 ==
  note: Must press during 1s
  Input : Inport
  AIR + : CoderSF_BSW_Libs/Digital I//O/Switch Output  Commented=on  channel=HSO03
  AIR +1 : CoderSF_BSW_Libs/Digital I//O/Switch Output  Commented=on  channel=HSO03
  AIR +2 : CoderSF_BSW_Libs/Digital I//O/Switch Output  channel=HSO04
  AIR - : CoderSF_BSW_Libs/Digital I//O/Switch Output  Commented=on  channel=HSO04
  AIR -1 : CoderSF_BSW_Libs/Digital I//O/Switch Output  channel=HSO03
  Cast To Boolean{,1..3} (4 alike) : DataTypeConversion  OutDataTypeStr=boolean
  Compare To Constant6 : simulink/Logic and Bit Operations/Compare To Constant  Commented=on  relop=>=  const=1  OutDataTypeStr=boolean
  Delay : Delay  DelayLength=1000
  Delay2 : Delay  DelayLength=1000
  Desabling inverter : Subsystem
  Detect Change : simulink/Logic and Bit Operations/Detect Change  Commented=on  vinit=0  OutDataTypeStr=boolean
  Discrete-Time Integrator3 : DiscreteIntegrator  Commented=on  ExternalReset=falling  SampleTime=-1  OutDataTypeStr=Inherit: Inherit via back propagation  UpperSaturationLimit=12  ICPrevOutput=DiscIntNeverNeededParam  ICPrevScaledInput=DiscIntNeverNeededParam
  Décharge ! : CoderSF_BSW_Libs/Digital I//O/Switch Output  channel=HSO08
  Enable Inverter : Subsystem  Commented=on
  Ground : Ground  Commented=on
  Logical Operator{,1..4,6} (6 alike) : Logic  Commented=on  Operator=NOT  IconShape=distinctive  AllPortsSameDT=off  OutDataTypeStr=boolean
  NOT : Logic  Operator=NOT  IconShape=distinctive  AllPortsSameDT=off  OutDataTypeStr=boolean
  NOT1 : Logic  Operator=NOT  IconShape=distinctive  AllPortsSameDT=off  OutDataTypeStr=boolean
  Precharge Relay : CoderSF_BSW_Libs/Digital I//O/Switch Output  Commented=on  channel=HSO05
  Precharge Relay1 : CoderSF_BSW_Libs/Digital I//O/Switch Output  channel=HSO05
  Read NVM : CoderSF_BSW_Libs/Non-volatile Memory Blocks/Read NVM  Commented=on  variable_name=nvmVdc_bus_V  variable_type=Inherit from 'Variable definition'
  Switch : Switch  Commented=on  Threshold=1
  Write Measurement1 : CoderSF_BSW_Libs/Calibration & Measurement/Write Measurement  Commented=on  variable_name=PRE  variable_value=0  variable_type=boolean  numD=1  unitStr=""  descStr=""
      settings: AttributesFormatString=type:%<variable_type> Dimensions:%<numD>
  Write Measurement2 : CoderSF_BSW_Libs/Calibration & Measurement/Write Measurement  Commented=on  variable_name=AIR_plus  variable_value=0  variable_type=boolean  numD=1  unitStr=""  descStr=""
      settings: AttributesFormatString=type:%<variable_type> Dimensions:%<numD>
  Write Measurement3 : CoderSF_BSW_Libs/Calibration & Measurement/Write Measurement  Commented=on  variable_name=AIR_moins  variable_value=0  variable_type=boolean  numD=1  unitStr=""  descStr=""
      settings: AttributesFormatString=type:%<variable_type> Dimensions:%<numD>
  Write Measurement4 : CoderSF_BSW_Libs/Calibration & Measurement/Write Measurement  Commented=on  variable_name=AIR_plus  variable_value=0  variable_type=boolean  numD=1  unitStr=""  descStr=""
      settings: AttributesFormatString=type:%<variable_type> Dimensions:%<numD>
  Write Measurement5 : CoderSF_BSW_Libs/Calibration & Measurement/Write Measurement  variable_name=PRE  variable_value=0  variable_type=boolean  numD=1  unitStr=""  descStr=""
      settings: AttributesFormatString=type:%<variable_type> Dimensions:%<numD>
  Write Measurement6 : CoderSF_BSW_Libs/Calibration & Measurement/Write Measurement  variable_name=AIR_moins  variable_value=0  variable_type=boolean  numD=1  unitStr=""  descStr=""
      settings: AttributesFormatString=type:%<variable_type> Dimensions:%<numD>
  Write Measurement7 : CoderSF_BSW_Libs/Calibration & Measurement/Write Measurement  variable_name=AIR_plus  variable_value=0  variable_type=boolean  numD=1  unitStr=""  descStr=""
      settings: AttributesFormatString=type:%<variable_type> Dimensions:%<numD>
  Write Measurement9 : CoderSF_BSW_Libs/Calibration & Measurement/Write Measurement  variable_name=DECHARGE  variable_value=0  variable_type=boolean  numD=1  unitStr=""  descStr=""
      settings: AttributesFormatString=type:%<variable_type> Dimensions:%<numD>
  Activate Inverter1 : Outport
  wires:
  Discrete-Time Integrator3/1 -> Compare To Constant6/1
  Read NVM/1 -> Detect Change/1
  Logical Operator6/1 -> Discrete-Time Integrator3/1, Discrete-Time Integrator3/2
  Detect Change/1 -> Logical Operator6/1
  Ground/1 -> Switch/1
  Compare To Constant6/1 -> Logical Operator3/1, Switch/2
  Logical Operator/1 -> AIR -/1
  Switch/1 -> Logical Operator1/1
  Logical Operator2/1 -> Write Measurement3/1
  Logical Operator1/1 -> Precharge Relay/1, Write Measurement1/1
  Logical Operator3/1 -> Write Measurement2/1, AIR +/1
  Logical Operator4/1 -> Write Measurement4/1, AIR +1/1
  Cast To Boolean/1 -> Precharge Relay1/1, Write Measurement5/1
  Cast To Boolean1/1 -> AIR -1/1, Write Measurement6/1
  Cast To Boolean2/1 -> AIR +2/1, Write Measurement7/1
  Cast To Boolean3/1 -> Write Measurement9/1, Décharge !/1
  Delay/1 -> Delay2/1
  Delay2/1 -> Cast To Boolean1/1
  NOT1/1 -> Cast To Boolean3/1
  NOT/1 -> Desabling inverter/Trigger, Enable Inverter/Trigger, Delay/1, NOT1/1, Cast To Boolean2/1, Cast To Boolean/1
  Input/1 -> Logical Operator/1, Logical Operator2/1, Switch/3, Activate Inverter1/1, NOT/1, Logical Operator4/1
